simulink model "case30_pidv2"  (R2026a)
settings: Solver=ode4  StopTime=8  FixedStep=1e-3
values from neighbouring files (symbols this model uses):
  C = mkC(G, trip)    [case30_pidv2_check.m]    (also in chan_check_sl.m = struct('G', G, 'Pm0', P0.Pm0(:), 'lo', P0.Pm0(:) - 1, 'hi', ; run_matrix_sl.m = struct('G', G, 'Pm0', P0.Pm0(:), 'lo', lo, 'hi', hi, 'rate',; run_v13_sl.m = struct('G', G, 'Pm0', P0.Pm0(:), 'lo', lo, 'hi', hi, 'rate',; speed_probe_sl.m = struct('G', G, 'Pm0', P0.Pm0(:), 'lo', lo, 'hi', hi, 'rate',)
  P = load(fullfile(here, '..', '..', 'bus_30', 'case30_simulink_data.mat'))    [case30_pidv2_build.m]    (also in chan_check_sl.m = L.scenario_P(P0, B, Yr, Vr, 'line', 1, 1, 1.0, 1.5); run_matrix_sl.m = L.scenario_P(P0, B, Yr, Vr, typ, S.alpha(k), S.loc(k), S.tf(; run_v13_sl.m = L.scenario_P(P0, B, Yr, Vr, typ, a, lc, S.tf(k), S.tc(k)); speed_probe_sl.m = L.scenario_P(P0, B, Yr, Vr, typ, S.alpha(k), S.loc(k), S.tf()
settings Model: Creator=rnoor  LastModifiedBy=rnoor

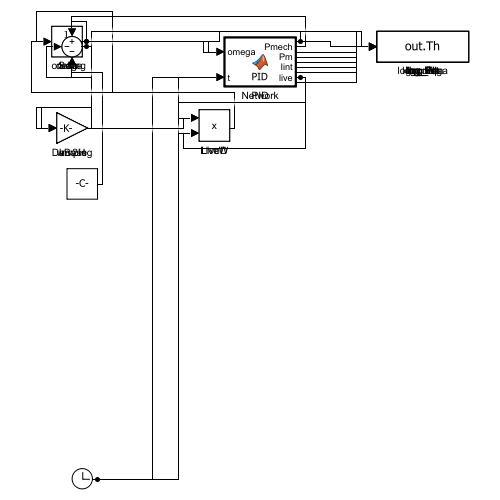
[thumbnail: Simulink's stored preview of the top-level diagram]
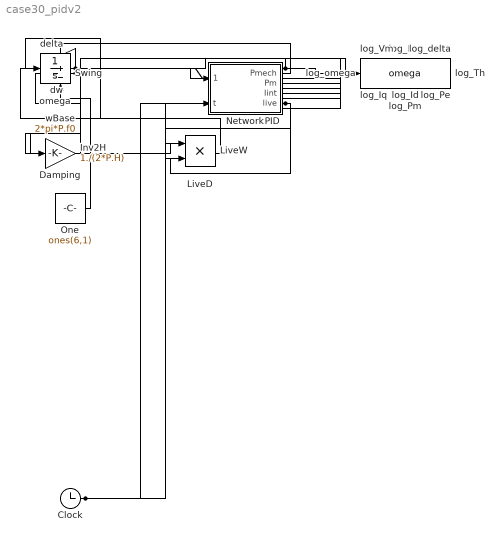
== system case30_pidv2 ==
  Clock : Clock
  Damping : Gain  Gain=P.D
  Inv2H : Gain  Gain=1./(2*P.H)
  LiveD : Product
  LiveW : Product
  Network : MATLAB Function  TreatAsAtomicUnit=on
  One : Constant  Value=ones(6,1)  VectorParams1D=off
  PID : MATLAB Function  TreatAsAtomicUnit=on  SystemSampleTime=1e-3
  Swing : Sum  Inputs=+--
  delta : Integrator  InitialCondition=P.delta0
  dw : Sum  Inputs=+-
  log_Id : ToWorkspace  VariableName=Id  SaveFormat=Timeseries  SampleTime=-1
  log_Iint : ToWorkspace  VariableName=Iint  SaveFormat=Timeseries  SampleTime=-1
  log_Iq : ToWorkspace  VariableName=Iq  SaveFormat=Timeseries  SampleTime=-1
  log_Pe : ToWorkspace  VariableName=Pe  SaveFormat=Timeseries  SampleTime=-1
  log_Pm : ToWorkspace  VariableName=Pm  SaveFormat=Timeseries  SampleTime=-1
  log_Th : ToWorkspace  VariableName=Th  SaveFormat=Timeseries  SampleTime=-1
  log_Vm : ToWorkspace  VariableName=Vm  SaveFormat=Timeseries  SampleTime=-1
  log_delta : ToWorkspace  VariableName=delta  SaveFormat=Timeseries  SampleTime=-1
  log_omega : ToWorkspace  VariableName=omega  SaveFormat=Timeseries  SampleTime=-1
  omega : Integrator  InitialCondition=ones(6,1)
  wBase : Gain  Gain=2*pi*P.f0
  wires:
  omega/1 -> dw/1, PID/1(omega), log_omega/1
  One/1 -> dw/2
  dw/1 -> wBase/1, Damping/1
  wBase/1 -> LiveD/1
  PID/4(live) -> LiveD/2, LiveW/2
  LiveD/1 -> delta/1
  PID/1(Pmech) -> Swing/1
  Network/1(Pe) -> Swing/2, log_Pe/1
  Damping/1 -> Swing/3
  Swing/1 -> Inv2H/1
  Inv2H/1 -> LiveW/1
  LiveW/1 -> omega/1
  delta/1 -> Network/1(delta), log_delta/1
  Clock/1 -> Network/2(t), PID/2(t)
  PID/2(Pm) -> log_Pm/1
  PID/3(Iint) -> log_Iint/1
  Network/2(Id) -> log_Id/1
  Network/3(Iq) -> log_Iq/1
  Network/4(Vm) -> log_Vm/1
  Network/5(Th) -> log_Th/1

== matlab function case30_pidv2/PID ==
  data: omega input; Pmech output; t input; Pm output; Iint output; live output; P parameter; C parameter
function [Pmech, Pm, Iint, live] = PID(omega, t, P, C)
persistent I xf pm
if isempty(I), I = C.Pm0; xf = zeros(size(C.Pm0)); pm = C.Pm0; end
tm = t + 0.5*C.h;
faulted = (tm >= P.t_fault) && (tm < P.t_clear);
k = min(floor((t + 1e-9) / C.Tl) + 1, size(C.G, 1));
Kp = reshape(C.G(k, :, 1), [], 1);  Ki = reshape(C.G(k, :, 2), [], 1);  Kd = reshape(C.G(k, :, 3), [], 1);
e = 1 - omega(:);
dterm = C.Nd * (e - xf);
xf_n = xf + C.h * C.Nd * (e - xf);
I_n = min(max(I + C.h * Ki .* e, C.lo), C.hi);
Ps = min(max(Kp .* e + I_n + Kd .* dterm, C.lo), C.hi);
pm_n = pm + min(max(Ps - pm, -C.rate * C.h), C.rate * C.h);
fz = (C.freeze > 0) & faulted;
xf(~fz) = xf_n(~fz);  I(~fz) = I_n(~fz);  pm(~fz) = pm_n(~fz);
Pmech = pm - C.trip * double(faulted);
Pm = pm;  Iint = I;  live = 1 - double((C.dead > 0) & faulted);
end

== matlab function case30_pidv2/Network ==
  data: delta input; Pe output; t input; Id output; Iq output; Vm output; Th output; P parameter
function [Pe, Id, Iq, Vm, Th] = Network(delta, t, P)
if t < P.t_fault - 1e-9
    Yr = P.Yred_pre;   Vr = P.Vrec_pre;
elseif t < P.t_clear - 1e-9
    Yr = P.Yred_fault; Vr = P.Vrec_fault;
else
    Yr = P.Yred_post;  Vr = P.Vrec_post;
end
rot = exp(1j*(delta(:) - pi/2));
E = (P.Ed + 1j*P.Eq) .* rot;
I = Yr * E;
Pe = real(E .* conj(I));
Idq = I ./ rot;
Id = real(Idq);  Iq = imag(Idq);
V = Vr * E;
Vm = abs(V);  Th = angle(V);
end
